simulink model "sschdlexSolarInverterSingleNetworkModel"  (R2026a)
settings: Solver=FixedStepDiscrete  StopTime=.5  MaxStep=1e-4
PreLoadFcn:
  | load('EmulatedPV_LowPowerData.mat');
  | irr = 0.15;
  | numIrr = 10;
  | ArrayPower = ArrayCurrent.*ArrayVoltage;
  | 
  | C_Boost_In = 680e-6;
  | C_Boost_In_R = 0;
  | L_Boost = 100e-6;
  | L_Boost_R = 0;
  | C_Boost_Out = 1640e-6;
  | 
  | TsFPGA = 2e-6;
  | TsControl = 2e-6;
  | TsCPU = 2e-6;
  | Tc = TsControl;
  | Ts = 2e-6;
  | 
  | IGBT_Vth = 6;
  | IGBT_Vf = 0.8;
  | IGBT_R = 0.001;
  | IGBT_Con = 1e-5;
  | 
  | IGBT_D_Vth = 0.8;
  | IGBT_D_R = 0.001;
  | IGBT_D_Con = 1e-5;
  | 
  | maxIn = 10;
  | minIn = -10;
  | maxOut = 2^15;
  | minOut = -2^15;
  | difIn = maxIn-minIn;
  | difOut = maxOut-minOut;
  | gain = difOut/difIn;
  | dc1 = (maxOut+minOut)/2;
  | dc2 = (maxIn+minIn)/2;
  | offset = dc1-gain*dc2;
  | numIrr = 10;
  | ArrayPower = ArrayCurrent.*ArrayVoltage;
InitFcn:
  | Ts = 2e-6;
  | Tc = Ts;
values from neighbouring files (symbols this model uses):
  ArrayCurrent = [3 2.90135967378 2.78442846347 2.64406556825 2.47269969012 2.25842875672 1.98100825201 1.60223040661 1.04533074246 0.222841716608 0 0 ... (1000 elements, 100x10)]    [EmulatedPV_LowPowerData.mat]
  ArrayVoltage = [0 0.151515151515 0.30303030303 0.454545454545 0.606060606061 0.757575757576 0.909090909091 1.06060606061 1.21212121212 1.36363636364 1.51515151515 1.66666666667 ... (100 elements, 100x1)]    [EmulatedPV_LowPowerData.mat]
  Irradiance = [0.05 0.1 0.15 0.2 0.25 0.3 0.35 0.4 0.45 0.5]    [EmulatedPV_LowPowerData.mat]
undefined symbols (not defined in the file or in its folder): DiscIntNeverNeededParam, ee_sli_rtmsupport, gcbh, Tdata
libraries: fl_lib x19, nesl_utility x12, eeGeneralControl x8, ee_lib x6, simulink x3, slpidlib x2
(part 2 of 2)

== system sschdlexSolarInverterSingleNetworkModel/MPPT and Boost Controllers/PWM Generator (2-Level) ==
  ref : Inport  SampleTime=Ts
  Carrier counter : Subsystem  LoadFcn=ee_sli_rtmsupport( 'loadfcn', gcbh );  mask(Counter){CarrCount=Up-Down, Range=Range, Tper=Tper, Tdelay=Td, Ts=Ts}
      mask prompts: CarrCount "physmod:ee:library:comments:control:eeGeneralControl:CounterType_MP"; Range "physmod:ee:library:comments:control:eeGeneralControl:OutputRange_MP"; Tper "physmod:ee:library:comments:control:eeGeneralControl:TimerPeriods_MP"; Tdelay "physmod:ee:library:comments:control:eeGeneralControl:PhaseDelays_MP"; Ts "physmod:ee:library:comments:control:eeGeneralControl:SampleTime_MP"
      mask help: physmod:ee:library:comments:control:eeGeneralControl:Counter_MD
      mask init:
      | timeDomain = ee.mask.getTimeDomain(Ts);
      settings: CopyFcn=ee_sli_rtmsupport( 'copyfcn', gcbh );  DeleteFcn=ee_sli_rtmsupport( 'deletefcn', gcbh );  ModelCloseFcn=ee_sli_rtmsupport( 'modelclosefcn', gcbh );  PostSaveFcn=ee_sli_rtmsupport( 'postsavefcn', gcbh );  PreCopyFcn=ee_sli_rtmsupport( 'precopyfcn', gcbh );  OpenFcn=ee_sli_rtmsupport( 'openfcn', gcbh );  CloseFcn=ee_sli_rtmsupport( 'closefcn', gcbh );  PreDeleteFcn=ee_sli_rtmsupport( 'predeletefcn', gcbh );
      mask Help: web(nesl_help(gcbh))
      mask TypeOptions CarrCount: physmod:ee:library:comments:control:eeGeneralControl:Up_PV | physmod:ee:library:comments:control:eeGeneralControl:Down_PV | physmod:ee:library:comments:control:eeGeneralControl:Up0x2DDown_PV
      mask TypeOptions Ts:
      | Integrator with
      | Wrapped State
      | (Discrete or Continuous)/Ts | Integrator with
      | Wrapped State
      | (Discrete or Continuous)1/Ts
      mask DialogControl ParameterGroupVar Prompt: physmod:ee:library:comments:control:eeGeneralControl:tab_Parameters
      mask DialogControl CarrCount Prompt: Counter type
      mask DialogControl Range Prompt: Output range
      mask DialogControl Tper Prompt: Timer period (s)
      mask DialogControl Tdelay Prompt: Phase delay (s)
      mask DialogControl Ts Prompt: Sample time
  Data Type Conversion2 : DataTypeConversion  SaturateOnIntegerOverflow=off  RndMeth=Floor
  Gain : Gain  Gain=-1
  Logical Operator : Logic  Operator=NOT  AllPortsSameDT=off  OutDataTypeStr=boolean
  Logical Operator1 : Logic  Operator=NOT  AllPortsSameDT=off  OutDataTypeStr=boolean
  Mux : Mux
  Relational Operator : RelationalOperator  OutDataTypeStr=boolean  RndMeth=Simplest  InputSameDT=off
  Relational Operator1 : RelationalOperator  OutDataTypeStr=boolean  RndMeth=Simplest  InputSameDT=off
  Selector : Selector  InputPortWidth=4  IndexOptions=Index vector (dialog)  Indices=PwmOutSelect  OutputSizes=1
  PWM : Outport  VectorParamsAs1DForOutWhenUnconnected=off
  wires:
  Relational Operator1/1 -> Mux/3, Logical Operator1/1
  Data Type Conversion2/1 -> PWM/1
  Relational Operator/1 -> Mux/1, Logical Operator/1
  Gain/1 -> Relational Operator1/1
  Logical Operator1/1 -> Mux/4
  Logical Operator/1 -> Mux/2
  Mux/1 -> Selector/1
  Carrier counter/1(T) -> Relational Operator1/2, Relational Operator/2
  ref/1 -> Gain/1, Relational Operator/1
  Selector/1 -> Data Type Conversion2/1

== system sschdlexSolarInverterSingleNetworkModel/MPPT and Boost Controllers/Perturb and Observe MPPT ==
  V : Inport
  I : Inport  Port=2
  VrefCmd : Inport  Port=3
  MPPT : Inport  Port=4
  delV : Inport  Port=5
  event : TriggerPort  VariantControl=(inherit)  ShowOutputPort=on
  " Demux " : Demux  Outputs=1
      settings: DisplayOption=none
  " SFunction " : S-Function  Tag=Stateflow S-Function 3  FunctionName=sf_sfun  PortCounts=[6 2]  SFunctionDeploymentMode=off  EnableBusSupport=on
  " Terminator " : Terminator
  Vref : Outport  VectorParamsAs1DForOutWhenUnconnected=off
  wires:
  V/1 -> " SFunction "/1
  I/1 -> " SFunction "/2
  VrefCmd/1 -> " SFunction "/3
  MPPT/1 -> " SFunction "/4
  delV/1 -> " SFunction "/5
  " SFunction "/2 -> Vref/1  "Vref"
  event/1 -> " SFunction "/6
  " Demux "/1 -> " Terminator "/1
  " SFunction "/1 -> " Demux "/1

== system sschdlexSolarInverterSingleNetworkModel/Open Loop Sweep1/PWM Generator (2-Level) ==
  ref : Inport  SampleTime=Ts
  Carrier counter : Subsystem  LoadFcn=ee_sli_rtmsupport( 'loadfcn', gcbh );  mask(Counter){CarrCount=Up-Down, Range=Range, Tper=Tper, Tdelay=Td, Ts=Ts}
      mask prompts: CarrCount "physmod:ee:library:comments:control:eeGeneralControl:CounterType_MP"; Range "physmod:ee:library:comments:control:eeGeneralControl:OutputRange_MP"; Tper "physmod:ee:library:comments:control:eeGeneralControl:TimerPeriods_MP"; Tdelay "physmod:ee:library:comments:control:eeGeneralControl:PhaseDelays_MP"; Ts "physmod:ee:library:comments:control:eeGeneralControl:SampleTime_MP"
      mask help: physmod:ee:library:comments:control:eeGeneralControl:Counter_MD
      mask init:
      | timeDomain = ee.mask.getTimeDomain(Ts);
      settings: CopyFcn=ee_sli_rtmsupport( 'copyfcn', gcbh );  DeleteFcn=ee_sli_rtmsupport( 'deletefcn', gcbh );  ModelCloseFcn=ee_sli_rtmsupport( 'modelclosefcn', gcbh );  PostSaveFcn=ee_sli_rtmsupport( 'postsavefcn', gcbh );  PreCopyFcn=ee_sli_rtmsupport( 'precopyfcn', gcbh );  OpenFcn=ee_sli_rtmsupport( 'openfcn', gcbh );  CloseFcn=ee_sli_rtmsupport( 'closefcn', gcbh );  PreDeleteFcn=ee_sli_rtmsupport( 'predeletefcn', gcbh );
      mask Help: web(nesl_help(gcbh))
      mask TypeOptions CarrCount: physmod:ee:library:comments:control:eeGeneralControl:Up_PV | physmod:ee:library:comments:control:eeGeneralControl:Down_PV | physmod:ee:library:comments:control:eeGeneralControl:Up0x2DDown_PV
      mask TypeOptions Ts:
      | Integrator with
      | Wrapped State
      | (Discrete or Continuous)/Ts | Integrator with
      | Wrapped State
      | (Discrete or Continuous)1/Ts
      mask DialogControl ParameterGroupVar Prompt: physmod:ee:library:comments:control:eeGeneralControl:tab_Parameters
      mask DialogControl CarrCount Prompt: Counter type
      mask DialogControl Range Prompt: Output range
      mask DialogControl Tper Prompt: Timer period (s)
      mask DialogControl Tdelay Prompt: Phase delay (s)
      mask DialogControl Ts Prompt: Sample time
  Data Type Conversion2 : DataTypeConversion  SaturateOnIntegerOverflow=off  RndMeth=Floor
  Gain : Gain  Gain=-1
  Logical Operator : Logic  Operator=NOT  AllPortsSameDT=off  OutDataTypeStr=boolean
  Logical Operator1 : Logic  Operator=NOT  AllPortsSameDT=off  OutDataTypeStr=boolean
  Mux : Mux
  Relational Operator : RelationalOperator  OutDataTypeStr=boolean  RndMeth=Simplest  InputSameDT=off
  Relational Operator1 : RelationalOperator  OutDataTypeStr=boolean  RndMeth=Simplest  InputSameDT=off
  Selector : Selector  InputPortWidth=4  IndexOptions=Index vector (dialog)  Indices=PwmOutSelect  OutputSizes=1
  PWM : Outport  VectorParamsAs1DForOutWhenUnconnected=off
  wires:
  Relational Operator1/1 -> Mux/3, Logical Operator1/1
  Data Type Conversion2/1 -> PWM/1
  Relational Operator/1 -> Mux/1, Logical Operator/1
  Gain/1 -> Relational Operator1/1
  Logical Operator1/1 -> Mux/4
  Logical Operator/1 -> Mux/2
  Mux/1 -> Selector/1
  Carrier counter/1(T) -> Relational Operator1/2, Relational Operator/2
  ref/1 -> Gain/1, Relational Operator/1
  Selector/1 -> Data Type Conversion2/1

== system sschdlexSolarInverterSingleNetworkModel/Open Loop Sweep2/PWM Generator (2-Level) ==
  ref : Inport  SampleTime=Ts
  Carrier counter : Subsystem  LoadFcn=ee_sli_rtmsupport( 'loadfcn', gcbh );  mask(Counter){CarrCount=Up-Down, Range=Range, Tper=Tper, Tdelay=Td, Ts=Ts}
      mask prompts: CarrCount "physmod:ee:library:comments:control:eeGeneralControl:CounterType_MP"; Range "physmod:ee:library:comments:control:eeGeneralControl:OutputRange_MP"; Tper "physmod:ee:library:comments:control:eeGeneralControl:TimerPeriods_MP"; Tdelay "physmod:ee:library:comments:control:eeGeneralControl:PhaseDelays_MP"; Ts "physmod:ee:library:comments:control:eeGeneralControl:SampleTime_MP"
      mask help: physmod:ee:library:comments:control:eeGeneralControl:Counter_MD
      mask init:
      | timeDomain = ee.mask.getTimeDomain(Ts);
      settings: CopyFcn=ee_sli_rtmsupport( 'copyfcn', gcbh );  DeleteFcn=ee_sli_rtmsupport( 'deletefcn', gcbh );  ModelCloseFcn=ee_sli_rtmsupport( 'modelclosefcn', gcbh );  PostSaveFcn=ee_sli_rtmsupport( 'postsavefcn', gcbh );  PreCopyFcn=ee_sli_rtmsupport( 'precopyfcn', gcbh );  OpenFcn=ee_sli_rtmsupport( 'openfcn', gcbh );  CloseFcn=ee_sli_rtmsupport( 'closefcn', gcbh );  PreDeleteFcn=ee_sli_rtmsupport( 'predeletefcn', gcbh );
      mask Help: web(nesl_help(gcbh))
      mask TypeOptions CarrCount: physmod:ee:library:comments:control:eeGeneralControl:Up_PV | physmod:ee:library:comments:control:eeGeneralControl:Down_PV | physmod:ee:library:comments:control:eeGeneralControl:Up0x2DDown_PV
      mask TypeOptions Ts:
      | Integrator with
      | Wrapped State
      | (Discrete or Continuous)/Ts | Integrator with
      | Wrapped State
      | (Discrete or Continuous)1/Ts
      mask DialogControl ParameterGroupVar Prompt: physmod:ee:library:comments:control:eeGeneralControl:tab_Parameters
      mask DialogControl CarrCount Prompt: Counter type
      mask DialogControl Range Prompt: Output range
      mask DialogControl Tper Prompt: Timer period (s)
      mask DialogControl Tdelay Prompt: Phase delay (s)
      mask DialogControl Ts Prompt: Sample time
  Data Type Conversion2 : DataTypeConversion  SaturateOnIntegerOverflow=off  RndMeth=Floor
  Gain : Gain  Gain=-1
  Logical Operator : Logic  Operator=NOT  AllPortsSameDT=off  OutDataTypeStr=boolean
  Logical Operator1 : Logic  Operator=NOT  AllPortsSameDT=off  OutDataTypeStr=boolean
  Mux : Mux
  Relational Operator : RelationalOperator  OutDataTypeStr=boolean  RndMeth=Simplest  InputSameDT=off
  Relational Operator1 : RelationalOperator  OutDataTypeStr=boolean  RndMeth=Simplest  InputSameDT=off
  Selector : Selector  InputPortWidth=4  IndexOptions=Index vector (dialog)  Indices=PwmOutSelect  OutputSizes=1
  PWM : Outport  VectorParamsAs1DForOutWhenUnconnected=off
  wires:
  Relational Operator1/1 -> Mux/3, Logical Operator1/1
  Data Type Conversion2/1 -> PWM/1
  Relational Operator/1 -> Mux/1, Logical Operator/1
  Gain/1 -> Relational Operator1/1
  Logical Operator1/1 -> Mux/4
  Logical Operator/1 -> Mux/2
  Mux/1 -> Selector/1
  Carrier counter/1(T) -> Relational Operator1/2, Relational Operator/2
  ref/1 -> Gain/1, Relational Operator/1
  Selector/1 -> Data Type Conversion2/1

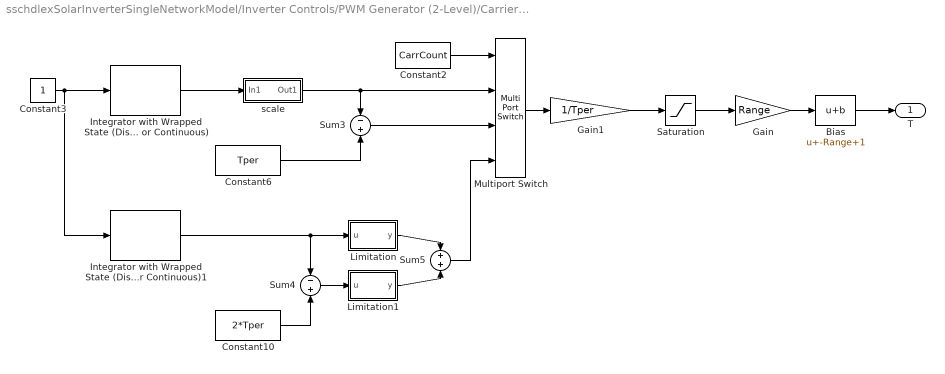
== system sschdlexSolarInverterSingleNetworkModel/Inverter Controls/PWM Generator (2-Level)/Carrier counter ==
  Bias : Bias  Bias=-Range+1  SaturateOnIntegerOverflow=off
  Constant10 : Constant  Value=2*Tper  SampleTime=Ts
  Constant2 : Constant  Value=CarrCount  SampleTime=Ts
  Constant3 : Constant  SampleTime=Ts
  Constant6 : Constant  Value=Tper  SampleTime=Ts
  Gain : Gain  Gain=Range
  Gain1 : Gain  Gain=1/Tper
  Integrator with Wrapped State (Discrete or Continuous) : eeGeneralControl/Integrator with Wrapped State (Discrete or Continuous)  LabelModeActiveChoice=Discrete  WrappedStateUpperValue=Tper  WrappedStateLowerValue=0  x0=min(Tdelay,Tper)  Ts=Ts
  Integrator with Wrapped State (Discrete or Continuous)1 : eeGeneralControl/Integrator with Wrapped State (Discrete or Continuous)  LabelModeActiveChoice=Discrete  WrappedStateUpperValue=2*Tper  WrappedStateLowerValue=0  x0=Tdelay  Ts=Ts
  Limitation : Subsystem
  Limitation1 : Subsystem
  Multiport Switch : MultiPortSwitch  SaturateOnIntegerOverflow=off  InputSameDT=off
  Saturation : Saturate  UpperLimit=1  LowerLimit=0
  Sum3 : Sum  Inputs=-+
  Sum4 : Sum  Inputs=-+
  Sum5 : Sum
  scale : Subsystem
  T : Outport  VectorParamsAs1DForOutWhenUnconnected=off
  wires:
  Integrator with Wrapped State (Discrete or Continuous)/1 -> scale/1(In1)
  Integrator with Wrapped State (Discrete or Continuous)1/1 -> Limitation/1(u), Sum4/1
  Multiport Switch/1 -> Gain1/1
  Constant3/1 -> Integrator with Wrapped State (Discrete or Continuous)1/1, Integrator with Wrapped State (Discrete or Continuous)/1
  Sum3/1 -> Multiport Switch/3
  Constant10/1 -> Sum4/2
  Limitation/1(y) -> Sum5/1
  Sum5/1 -> Multiport Switch/4
  scale/1(Out1) -> Multiport Switch/2, Sum3/1
  Limitation1/1(y) -> Sum5/2
  Constant6/1 -> Sum3/2
  Sum4/1 -> Limitation1/1(u)
  Constant2/1 -> Multiport Switch/1
  Gain/1 -> Bias/1
  Gain1/1 -> Saturation/1
  Bias/1 -> T/1
  Saturation/1 -> Gain/1

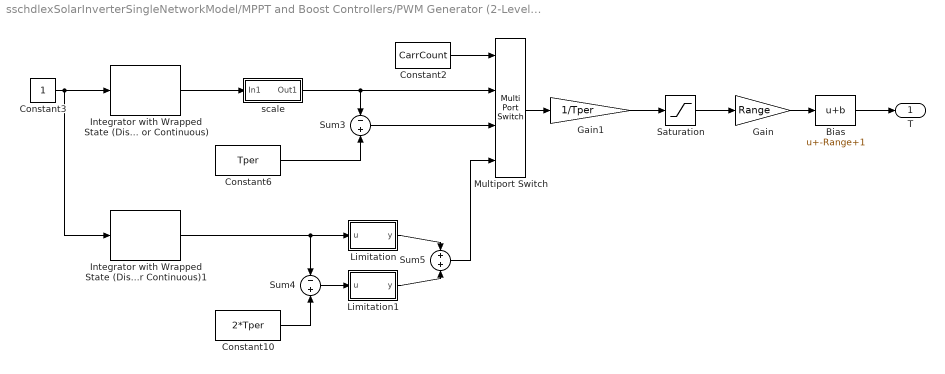
== system sschdlexSolarInverterSingleNetworkModel/MPPT and Boost Controllers/PWM Generator (2-Level)/Carrier counter ==
  Bias : Bias  Bias=-Range+1  SaturateOnIntegerOverflow=off
  Constant10 : Constant  Value=2*Tper  SampleTime=Ts
  Constant2 : Constant  Value=CarrCount  SampleTime=Ts
  Constant3 : Constant  SampleTime=Ts
  Constant6 : Constant  Value=Tper  SampleTime=Ts
  Gain : Gain  Gain=Range
  Gain1 : Gain  Gain=1/Tper
  Integrator with Wrapped State (Discrete or Continuous) : eeGeneralControl/Integrator with Wrapped State (Discrete or Continuous)  LabelModeActiveChoice=Discrete  WrappedStateUpperValue=Tper  WrappedStateLowerValue=0  x0=min(Tdelay,Tper)  Ts=Ts
  Integrator with Wrapped State (Discrete or Continuous)1 : eeGeneralControl/Integrator with Wrapped State (Discrete or Continuous)  LabelModeActiveChoice=Discrete  WrappedStateUpperValue=2*Tper  WrappedStateLowerValue=0  x0=Tdelay  Ts=Ts
  Limitation : Subsystem
  Limitation1 : Subsystem
  Multiport Switch : MultiPortSwitch  SaturateOnIntegerOverflow=off  InputSameDT=off
  Saturation : Saturate  UpperLimit=1  LowerLimit=0
  Sum3 : Sum  Inputs=-+
  Sum4 : Sum  Inputs=-+
  Sum5 : Sum
  scale : Subsystem
  T : Outport  VectorParamsAs1DForOutWhenUnconnected=off
  wires:
  Integrator with Wrapped State (Discrete or Continuous)/1 -> scale/1(In1)
  Integrator with Wrapped State (Discrete or Continuous)1/1 -> Limitation/1(u), Sum4/1
  Multiport Switch/1 -> Gain1/1
  Constant3/1 -> Integrator with Wrapped State (Discrete or Continuous)1/1, Integrator with Wrapped State (Discrete or Continuous)/1
  Sum3/1 -> Multiport Switch/3
  Constant10/1 -> Sum4/2
  Limitation/1(y) -> Sum5/1
  Sum5/1 -> Multiport Switch/4
  scale/1(Out1) -> Multiport Switch/2, Sum3/1
  Limitation1/1(y) -> Sum5/2
  Constant6/1 -> Sum3/2
  Sum4/1 -> Limitation1/1(u)
  Constant2/1 -> Multiport Switch/1
  Gain/1 -> Bias/1
  Gain1/1 -> Saturation/1
  Bias/1 -> T/1
  Saturation/1 -> Gain/1

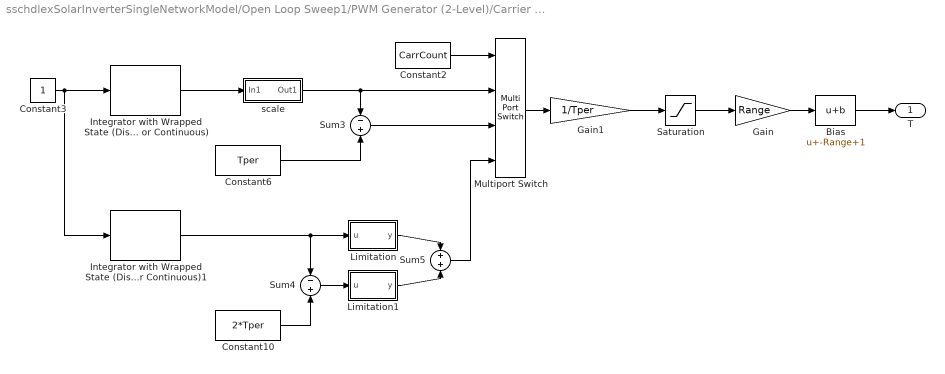
== system sschdlexSolarInverterSingleNetworkModel/Open Loop Sweep1/PWM Generator (2-Level)/Carrier counter ==
  Bias : Bias  Bias=-Range+1  SaturateOnIntegerOverflow=off
  Constant10 : Constant  Value=2*Tper  SampleTime=Ts
  Constant2 : Constant  Value=CarrCount  SampleTime=Ts
  Constant3 : Constant  SampleTime=Ts
  Constant6 : Constant  Value=Tper  SampleTime=Ts
  Gain : Gain  Gain=Range
  Gain1 : Gain  Gain=1/Tper
  Integrator with Wrapped State (Discrete or Continuous) : eeGeneralControl/Integrator with Wrapped State (Discrete or Continuous)  LabelModeActiveChoice=Discrete  WrappedStateUpperValue=Tper  WrappedStateLowerValue=0  x0=min(Tdelay,Tper)  Ts=Ts
  Integrator with Wrapped State (Discrete or Continuous)1 : eeGeneralControl/Integrator with Wrapped State (Discrete or Continuous)  LabelModeActiveChoice=Discrete  WrappedStateUpperValue=2*Tper  WrappedStateLowerValue=0  x0=Tdelay  Ts=Ts
  Limitation : Subsystem
  Limitation1 : Subsystem
  Multiport Switch : MultiPortSwitch  SaturateOnIntegerOverflow=off  InputSameDT=off
  Saturation : Saturate  UpperLimit=1  LowerLimit=0
  Sum3 : Sum  Inputs=-+
  Sum4 : Sum  Inputs=-+
  Sum5 : Sum
  scale : Subsystem
  T : Outport  VectorParamsAs1DForOutWhenUnconnected=off
  wires:
  Integrator with Wrapped State (Discrete or Continuous)/1 -> scale/1(In1)
  Integrator with Wrapped State (Discrete or Continuous)1/1 -> Limitation/1(u), Sum4/1
  Multiport Switch/1 -> Gain1/1
  Constant3/1 -> Integrator with Wrapped State (Discrete or Continuous)1/1, Integrator with Wrapped State (Discrete or Continuous)/1
  Sum3/1 -> Multiport Switch/3
  Constant10/1 -> Sum4/2
  Limitation/1(y) -> Sum5/1
  Sum5/1 -> Multiport Switch/4
  scale/1(Out1) -> Multiport Switch/2, Sum3/1
  Limitation1/1(y) -> Sum5/2
  Constant6/1 -> Sum3/2
  Sum4/1 -> Limitation1/1(u)
  Constant2/1 -> Multiport Switch/1
  Gain/1 -> Bias/1
  Gain1/1 -> Saturation/1
  Bias/1 -> T/1
  Saturation/1 -> Gain/1

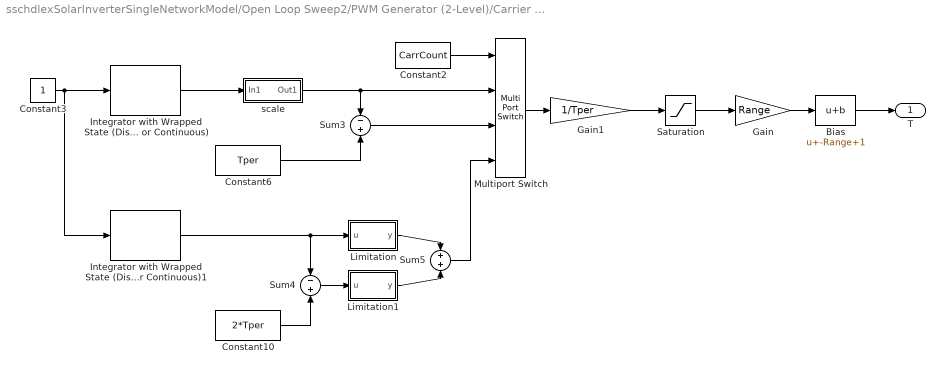
== system sschdlexSolarInverterSingleNetworkModel/Open Loop Sweep2/PWM Generator (2-Level)/Carrier counter ==
  Bias : Bias  Bias=-Range+1  SaturateOnIntegerOverflow=off
  Constant10 : Constant  Value=2*Tper  SampleTime=Ts
  Constant2 : Constant  Value=CarrCount  SampleTime=Ts
  Constant3 : Constant  SampleTime=Ts
  Constant6 : Constant  Value=Tper  SampleTime=Ts
  Gain : Gain  Gain=Range
  Gain1 : Gain  Gain=1/Tper
  Integrator with Wrapped State (Discrete or Continuous) : eeGeneralControl/Integrator with Wrapped State (Discrete or Continuous)  LabelModeActiveChoice=Discrete  WrappedStateUpperValue=Tper  WrappedStateLowerValue=0  x0=min(Tdelay,Tper)  Ts=Ts
  Integrator with Wrapped State (Discrete or Continuous)1 : eeGeneralControl/Integrator with Wrapped State (Discrete or Continuous)  LabelModeActiveChoice=Discrete  WrappedStateUpperValue=2*Tper  WrappedStateLowerValue=0  x0=Tdelay  Ts=Ts
  Limitation : Subsystem
  Limitation1 : Subsystem
  Multiport Switch : MultiPortSwitch  SaturateOnIntegerOverflow=off  InputSameDT=off
  Saturation : Saturate  UpperLimit=1  LowerLimit=0
  Sum3 : Sum  Inputs=-+
  Sum4 : Sum  Inputs=-+
  Sum5 : Sum
  scale : Subsystem
  T : Outport  VectorParamsAs1DForOutWhenUnconnected=off
  wires:
  Integrator with Wrapped State (Discrete or Continuous)/1 -> scale/1(In1)
  Integrator with Wrapped State (Discrete or Continuous)1/1 -> Limitation/1(u), Sum4/1
  Multiport Switch/1 -> Gain1/1
  Constant3/1 -> Integrator with Wrapped State (Discrete or Continuous)1/1, Integrator with Wrapped State (Discrete or Continuous)/1
  Sum3/1 -> Multiport Switch/3
  Constant10/1 -> Sum4/2
  Limitation/1(y) -> Sum5/1
  Sum5/1 -> Multiport Switch/4
  scale/1(Out1) -> Multiport Switch/2, Sum3/1
  Limitation1/1(y) -> Sum5/2
  Constant6/1 -> Sum3/2
  Sum4/1 -> Limitation1/1(u)
  Constant2/1 -> Multiport Switch/1
  Gain/1 -> Bias/1
  Gain1/1 -> Saturation/1
  Bias/1 -> T/1
  Saturation/1 -> Gain/1

== system sschdlexSolarInverterSingleNetworkModel/Inverter Controls/PWM Generator (2-Level)/Carrier counter/Limitation ==
  u : Inport
  Constant2 : Constant  Value=0  SampleTime=Ts
  Switch : Switch  Criteria=u2 > Threshold  Threshold=Tper  SaturateOnIntegerOverflow=off  InputSameDT=off
  y : Outport  VectorParamsAs1DForOutWhenUnconnected=off
  wires:
  u/1 -> Switch/2, Switch/3
  Switch/1 -> y/1
  Constant2/1 -> Switch/1

== system sschdlexSolarInverterSingleNetworkModel/Inverter Controls/PWM Generator (2-Level)/Carrier counter/Limitation1 ==
  u : Inport
  Constant2 : Constant  Value=0  SampleTime=Ts
  Switch : Switch  Criteria=u2 > Threshold  Threshold=Tper  SaturateOnIntegerOverflow=off  InputSameDT=off
  y : Outport  VectorParamsAs1DForOutWhenUnconnected=off
  wires:
  Constant2/1 -> Switch/1
  Switch/1 -> y/1
  u/1 -> Switch/3, Switch/2

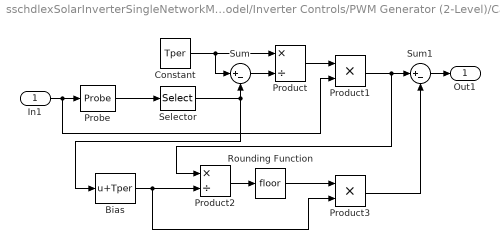
== system sschdlexSolarInverterSingleNetworkModel/Inverter Controls/PWM Generator (2-Level)/Carrier counter/scale ==
  In1 : Inport
  Bias : Bias  Bias=Tper  SaturateOnIntegerOverflow=off
  Constant : Constant  Value=Tper  SampleTime=Ts
  Probe : Probe  ProbeWidth=off  ProbeComplexSignal=off
  Product : Product  Inputs=*/
  Product1 : Product
  Product2 : Product  Inputs=*/
  Product3 : Product
  Rounding Function : Rounding
  Selector : Selector  InputPortWidth=2  IndexOptions=Index vector (dialog)  Indices=1  OutputSizes=1
  Sum : Sum  Inputs=|+-
  Sum1 : Sum  Inputs=|+-
  Out1 : Outport  VectorParamsAs1DForOutWhenUnconnected=off
  wires:
  Probe/1 -> Selector/1
  In1/1 -> Product1/2, Probe/1
  Selector/1 -> Bias/1, Sum/2
  Constant/1 -> Sum/1, Product/1
  Sum/1 -> Product/2
  Product/1 -> Product1/1
  Product1/1 -> Sum1/1, Product2/1
  Bias/1 -> Product3/2, Product2/2
  Product2/1 -> Rounding Function/1
  Rounding Function/1 -> Product3/1
  Sum1/1 -> Out1/1
  Product3/1 -> Sum1/2

== system sschdlexSolarInverterSingleNetworkModel/MPPT and Boost Controllers/PWM Generator (2-Level)/Carrier counter/Limitation ==
  u : Inport
  Constant2 : Constant  Value=0  SampleTime=Ts
  Switch : Switch  Criteria=u2 > Threshold  Threshold=Tper  SaturateOnIntegerOverflow=off  InputSameDT=off
  y : Outport  VectorParamsAs1DForOutWhenUnconnected=off
  wires:
  u/1 -> Switch/2, Switch/3
  Switch/1 -> y/1
  Constant2/1 -> Switch/1

== system sschdlexSolarInverterSingleNetworkModel/MPPT and Boost Controllers/PWM Generator (2-Level)/Carrier counter/Limitation1 ==
  u : Inport
  Constant2 : Constant  Value=0  SampleTime=Ts
  Switch : Switch  Criteria=u2 > Threshold  Threshold=Tper  SaturateOnIntegerOverflow=off  InputSameDT=off
  y : Outport  VectorParamsAs1DForOutWhenUnconnected=off
  wires:
  Constant2/1 -> Switch/1
  Switch/1 -> y/1
  u/1 -> Switch/3, Switch/2

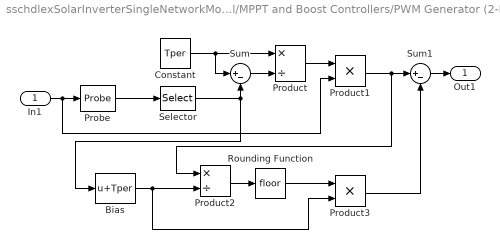
== system sschdlexSolarInverterSingleNetworkModel/MPPT and Boost Controllers/PWM Generator (2-Level)/Carrier counter/scale ==
  In1 : Inport
  Bias : Bias  Bias=Tper  SaturateOnIntegerOverflow=off
  Constant : Constant  Value=Tper  SampleTime=Ts
  Probe : Probe  ProbeWidth=off  ProbeComplexSignal=off
  Product : Product  Inputs=*/
  Product1 : Product
  Product2 : Product  Inputs=*/
  Product3 : Product
  Rounding Function : Rounding
  Selector : Selector  InputPortWidth=2  IndexOptions=Index vector (dialog)  Indices=1  OutputSizes=1
  Sum : Sum  Inputs=|+-
  Sum1 : Sum  Inputs=|+-
  Out1 : Outport  VectorParamsAs1DForOutWhenUnconnected=off
  wires:
  Probe/1 -> Selector/1
  In1/1 -> Product1/2, Probe/1
  Selector/1 -> Bias/1, Sum/2
  Constant/1 -> Sum/1, Product/1
  Sum/1 -> Product/2
  Product/1 -> Product1/1
  Product1/1 -> Sum1/1, Product2/1
  Bias/1 -> Product3/2, Product2/2
  Product2/1 -> Rounding Function/1
  Rounding Function/1 -> Product3/1
  Sum1/1 -> Out1/1
  Product3/1 -> Sum1/2

== system sschdlexSolarInverterSingleNetworkModel/Open Loop Sweep1/PWM Generator (2-Level)/Carrier counter/Limitation ==
  u : Inport
  Constant2 : Constant  Value=0  SampleTime=Ts
  Switch : Switch  Criteria=u2 > Threshold  Threshold=Tper  SaturateOnIntegerOverflow=off  InputSameDT=off
  y : Outport  VectorParamsAs1DForOutWhenUnconnected=off
  wires:
  u/1 -> Switch/2, Switch/3
  Switch/1 -> y/1
  Constant2/1 -> Switch/1

== system sschdlexSolarInverterSingleNetworkModel/Open Loop Sweep1/PWM Generator (2-Level)/Carrier counter/Limitation1 ==
  u : Inport
  Constant2 : Constant  Value=0  SampleTime=Ts
  Switch : Switch  Criteria=u2 > Threshold  Threshold=Tper  SaturateOnIntegerOverflow=off  InputSameDT=off
  y : Outport  VectorParamsAs1DForOutWhenUnconnected=off
  wires:
  Constant2/1 -> Switch/1
  Switch/1 -> y/1
  u/1 -> Switch/3, Switch/2

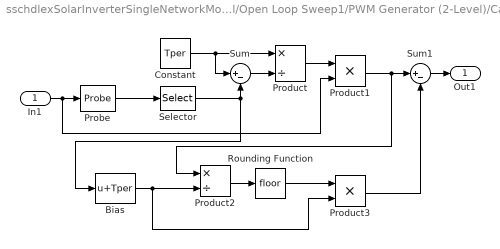
== system sschdlexSolarInverterSingleNetworkModel/Open Loop Sweep1/PWM Generator (2-Level)/Carrier counter/scale ==
  In1 : Inport
  Bias : Bias  Bias=Tper  SaturateOnIntegerOverflow=off
  Constant : Constant  Value=Tper  SampleTime=Ts
  Probe : Probe  ProbeWidth=off  ProbeComplexSignal=off
  Product : Product  Inputs=*/
  Product1 : Product
  Product2 : Product  Inputs=*/
  Product3 : Product
  Rounding Function : Rounding
  Selector : Selector  InputPortWidth=2  IndexOptions=Index vector (dialog)  Indices=1  OutputSizes=1
  Sum : Sum  Inputs=|+-
  Sum1 : Sum  Inputs=|+-
  Out1 : Outport  VectorParamsAs1DForOutWhenUnconnected=off
  wires:
  Probe/1 -> Selector/1
  In1/1 -> Product1/2, Probe/1
  Selector/1 -> Bias/1, Sum/2
  Constant/1 -> Sum/1, Product/1
  Sum/1 -> Product/2
  Product/1 -> Product1/1
  Product1/1 -> Sum1/1, Product2/1
  Bias/1 -> Product3/2, Product2/2
  Product2/1 -> Rounding Function/1
  Rounding Function/1 -> Product3/1
  Sum1/1 -> Out1/1
  Product3/1 -> Sum1/2

== system sschdlexSolarInverterSingleNetworkModel/Open Loop Sweep2/PWM Generator (2-Level)/Carrier counter/Limitation ==
  u : Inport
  Constant2 : Constant  Value=0  SampleTime=Ts
  Switch : Switch  Criteria=u2 > Threshold  Threshold=Tper  SaturateOnIntegerOverflow=off  InputSameDT=off
  y : Outport  VectorParamsAs1DForOutWhenUnconnected=off
  wires:
  u/1 -> Switch/2, Switch/3
  Switch/1 -> y/1
  Constant2/1 -> Switch/1

== system sschdlexSolarInverterSingleNetworkModel/Open Loop Sweep2/PWM Generator (2-Level)/Carrier counter/Limitation1 ==
  u : Inport
  Constant2 : Constant  Value=0  SampleTime=Ts
  Switch : Switch  Criteria=u2 > Threshold  Threshold=Tper  SaturateOnIntegerOverflow=off  InputSameDT=off
  y : Outport  VectorParamsAs1DForOutWhenUnconnected=off
  wires:
  Constant2/1 -> Switch/1
  Switch/1 -> y/1
  u/1 -> Switch/3, Switch/2

== system sschdlexSolarInverterSingleNetworkModel/Open Loop Sweep2/PWM Generator (2-Level)/Carrier counter/scale ==
  In1 : Inport
  Bias : Bias  Bias=Tper  SaturateOnIntegerOverflow=off
  Constant : Constant  Value=Tper  SampleTime=Ts
  Probe : Probe  ProbeWidth=off  ProbeComplexSignal=off
  Product : Product  Inputs=*/
  Product1 : Product
  Product2 : Product  Inputs=*/
  Product3 : Product
  Rounding Function : Rounding
  Selector : Selector  InputPortWidth=2  IndexOptions=Index vector (dialog)  Indices=1  OutputSizes=1
  Sum : Sum  Inputs=|+-
  Sum1 : Sum  Inputs=|+-
  Out1 : Outport  VectorParamsAs1DForOutWhenUnconnected=off
  wires:
  Probe/1 -> Selector/1
  In1/1 -> Product1/2, Probe/1
  Selector/1 -> Bias/1, Sum/2
  Constant/1 -> Sum/1, Product/1
  Sum/1 -> Product/2
  Product/1 -> Product1/1
  Product1/1 -> Sum1/1, Product2/1
  Bias/1 -> Product3/2, Product2/2
  Product2/1 -> Rounding Function/1
  Rounding Function/1 -> Product3/1
  Sum1/1 -> Out1/1
  Product3/1 -> Sum1/2
